simulink model "lab2_ea"  (R2026a)
settings: Solver=FixedStepAuto  FixedStep=0.001
model workspace (MAT data in the model file):
  k_1 = -1.81
  tau = 0.0231
settings Model: Creator=erica  LastModifiedBy=erica

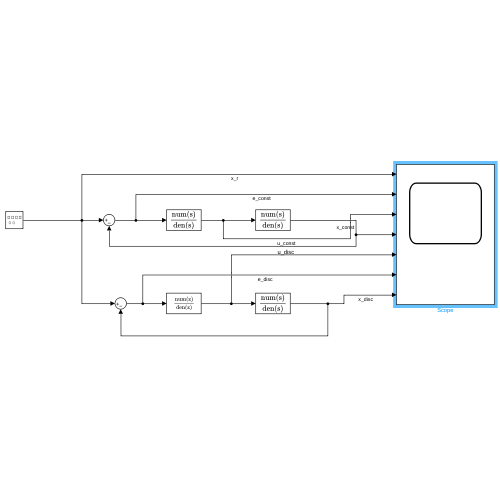
[thumbnail: Simulink's stored preview of the top-level diagram]
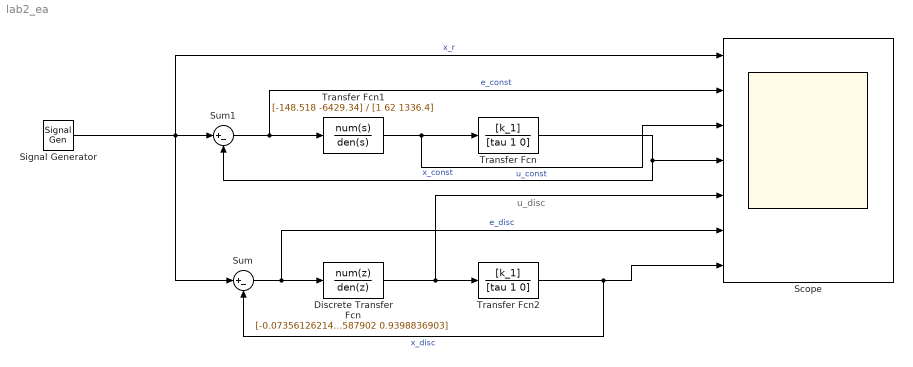
== system lab2_ea ==
  note: u_disc
  Discrete Transfer Fcn : DiscreteTransferFcn  Numerator=[-0.07356126214 -0.003117002633 0.07044425951]  Denominator=[1 -1.938587902 0.9398836903]
  Scope : Scope  NumInputPorts=7
      settings: ActiveDisplayYMinimum=-0.42897411330863  ActiveDisplayYMaximum=1.1365578014632378
  Signal Generator : SignalGenerator  WaveForm=square  Amplitude=0.7  Frequency=0.5
  Sum : Sum  Inputs=|+-
  Sum1 : Sum  Inputs=|+-
  Transfer Fcn : TransferFcn  Numerator=[k_1]  Denominator=[tau 1 0]
  Transfer Fcn1 : TransferFcn  Numerator=[-148.518 -6429.34]  Denominator=[1 62 1336.4]
  Transfer Fcn2 : TransferFcn  Numerator=[k_1]  Denominator=[tau 1 0]
  wires:
  Transfer Fcn1/1 -> Scope/3, Transfer Fcn/1  "u_const"
  Transfer Fcn/1 -> Sum1/2, Scope/4  "x_const"
  Signal Generator/1 -> Sum/1, Scope/1, Sum1/1  "x_r"
  Sum1/1 -> Scope/2, Transfer Fcn1/1  "e_const"
  Transfer Fcn2/1 -> Sum/2, Scope/7  "x_disc"
  Discrete Transfer Fcn/1 -> Scope/5, Transfer Fcn2/1
  Sum/1 -> Scope/6, Discrete Transfer Fcn/1  "e_disc"
